simulink model "lab2"  (R2024b)
settings: Solver=ode4  StartTime=0.0  StopTime=100.0  FixedStep=0.01  RelTol=1e-3
values from neighbouring files (symbols this model uses):
  A = [0 0 0; 1 0 -1; 0 1 2]    [main.m]
  Ac = J + H * F * M    [main.m]
  B = [0 -1; 1 0; 0 1]    [main.m]
  Bc = K + H * F * N    [main.m]
  C = [1 0 1]    [main.m]
  Fc = F * M    [main.m]
  Gc = F * N    [main.m]
settings Model: Creator=rober  LastModifiedBy=rober

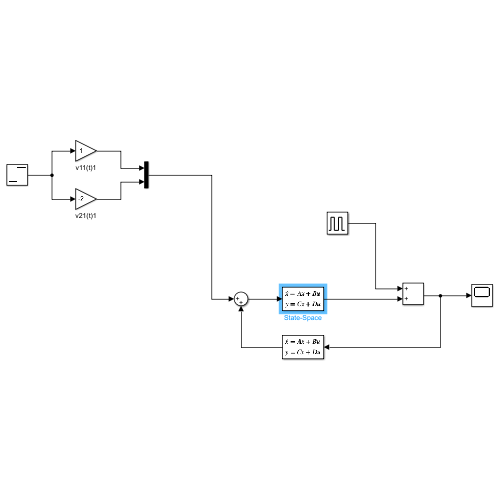
[thumbnail: Simulink's stored preview of the top-level diagram]
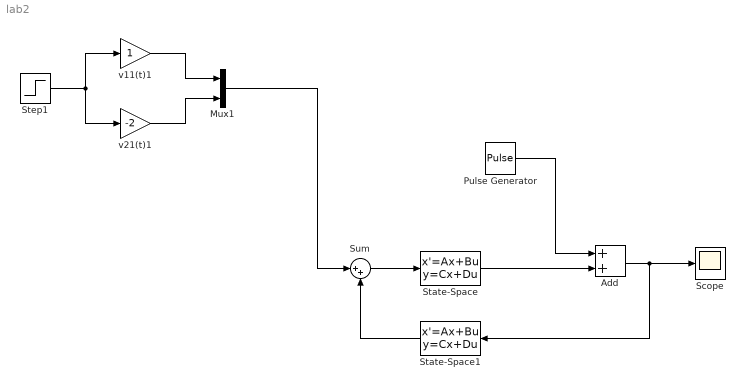
== system lab2 ==
  Add : Sum
  Mux1 : Mux  Inputs=2
  Pulse Generator : DiscretePulseGenerator  PulseType=Time based  Amplitude=0.01  Period=20  PulseWidth=5
  Scope : Scope
  State-Space : StateSpace  A=A  B=B  C=C  D=[0 0]  InitialCondition=0
  State-Space1 : StateSpace  A=Ac  B=Bc  C=Fc  D=Gc  InitialCondition=0
  Step1 : Step  SampleTime=0
  Sum : Sum  Inputs=|++
  v11(t)1 : Gain
  v21(t)1 : Gain  Gain=-2
  wires:
  Mux1/1 -> Sum/1
  Step1/1 -> v11(t)1/1, v21(t)1/1
  v11(t)1/1 -> Mux1/1
  v21(t)1/1 -> Mux1/2
  Sum/1 -> State-Space/1
  State-Space1/1 -> Sum/2
  State-Space/1 -> Add/2
  Add/1 -> Scope/1, State-Space1/1
  Pulse Generator/1 -> Add/1
